simulink model "DDMR_SS"  (R2024b)
settings: Solver=VariableStepAuto  StartTime=0.0  StopTime=30  RelTol=1e-3
values from neighbouring files (symbols this model uses):
  A_steer = [0, -V_ref; 0, 0]    [LQR.m]    (also in Track.m; Track2.m)
  B_steer = [0; 1]    [LQR.m]    (also in Track.m; Track2.m)
  K = lqr(A_full, B_full, Q_lqr, R_lqr)    [LQR.m]    (also in Track.m = [K_brake, 0, 0; Track2.m)
  L = 0.2    [LQR.m]    (also in Track.m; Track2.m)
  L_f = 0.2    [LQR.m]    (also in Track.m; Track2.m)
  L_obs = lqr(A_steer', C_steer', Q_obs, R_obs)'    [LQR.m]    (also in Track.m = place(A_steer', C_steer', poles_obs)'; Track2.m)
  line_width = 0.03    [LQR.m]    (also in Track.m; Track2.m)
  R = 0.05    [LQR.m]    (also in Track.m; Track2.m)
  track_pts = [2*cos(linspace(0, 2*pi, 1000)'), 2*sin(linspace(0, 2*pi, 1000)').*cos(linspace(0, 2*pi, 1000)')]    [LQR.m]    (also in Track.m; Track2.m = [track_pts; segments{i}])
  W_spread = 0.15    [LQR.m]    (also in Track.m; Track2.m)
settings Model: Creator=moham  LastModifiedBy=moham

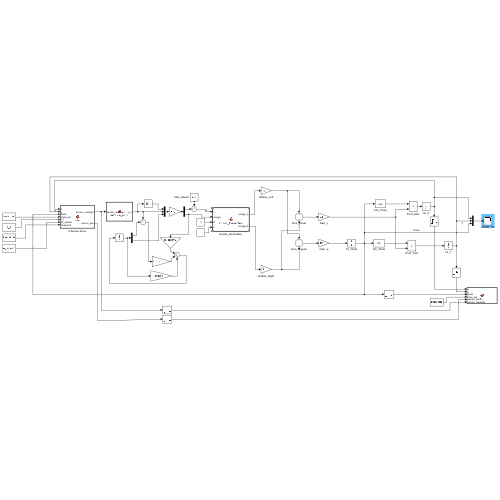
[thumbnail: Simulink's stored preview of the top-level diagram]
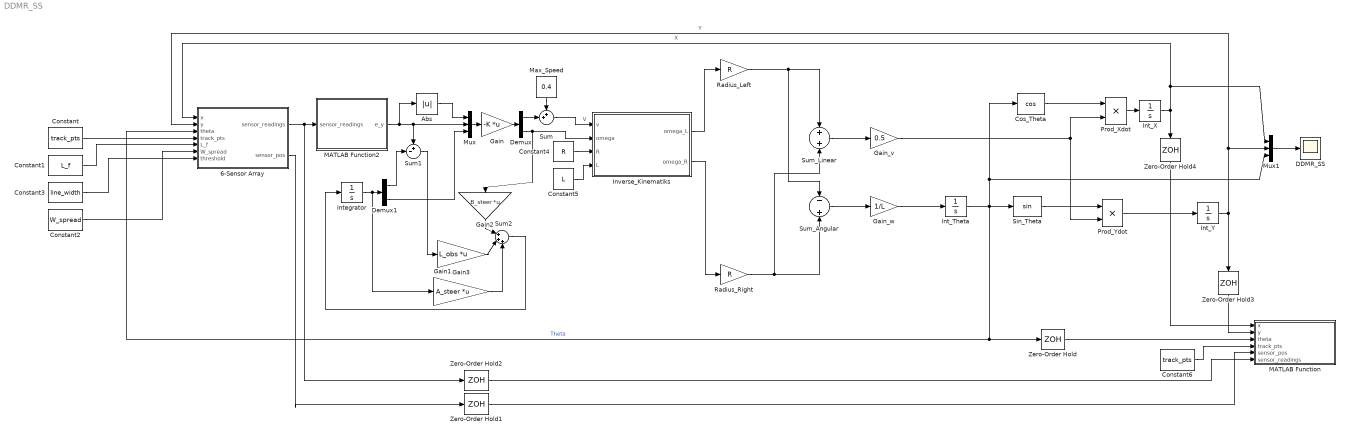
== system DDMR_SS ==
  6-Sensor Array : MATLAB Function  TreatAsAtomicUnit=on
  Abs : Abs  SaturateOnIntegerOverflow=off
  Constant : Constant  Value=track_pts
  Constant1 : Constant  Value=L_f
  Constant2 : Constant  Value=W_spread
  Constant3 : Constant  Value=line_width
  Constant4 : Constant  Value=R
  Constant5 : Constant  Value=L
  Constant6 : Constant  Value=track_pts
  Cos_Theta : Trigonometry  Operator=cos
  DDMR_SS : Scope
  Demux : Demux  Outputs=2
  Demux1 : Demux  Outputs=2
  Gain : Gain  Gain=-K  Multiplication=Matrix(K*u)
  Gain1 : Gain  Gain=A_steer  Multiplication=Matrix(K*u)
  Gain2 : Gain  Gain=B_steer  Multiplication=Matrix(K*u)
  Gain3 : Gain  Gain=L_obs  Multiplication=Matrix(K*u)
  Gain_v : Gain  Gain=0.5
  Gain_w : Gain  Gain=1/L
  Int_Theta : Integrator  InitialCondition=pi/-3
  Int_X : Integrator
  Int_Y : Integrator
  Integrator : Integrator  InitialCondition=[0; 0]
  "Inverse_Kinematiks " : MATLAB Function  TreatAsAtomicUnit=on
  MATLAB Function : MATLAB Function  TreatAsAtomicUnit=on
  MATLAB Function2 : MATLAB Function  TreatAsAtomicUnit=on
  Max_Speed : Constant  Value=0.4
  Mux : Mux  Inputs=3
  Mux1 : Mux  Inputs=3
  Prod_Xdot : Product
  Prod_Ydot : Product
  Radius_Left : Gain  Gain=R
  Radius_Right : Gain  Gain=R
  Sin_Theta : Trigonometry
  Sum : Sum  Inputs=++|
  Sum1 : Sum  Inputs=+-|
  Sum2 : Sum  Inputs=|+++
  Sum_Angular : Sum  Inputs=-+
  Sum_Linear : Sum
  Zero-Order Hold{,1..4} (5 alike) : ZeroOrderHold  SampleTime=0.033
  wires:
  "Inverse_Kinematiks "/1(omega_L) -> Radius_Left/1
  "Inverse_Kinematiks "/2(omega_R) -> Radius_Right/1
  Prod_Ydot/1 -> Int_Y/1
  Cos_Theta/1 -> Prod_Xdot/1
  Gain_v/1 -> Prod_Xdot/2, Prod_Ydot/2
  Sin_Theta/1 -> Prod_Ydot/1
  Prod_Xdot/1 -> Int_X/1
  Gain_w/1 -> Int_Theta/1
  Radius_Left/1 -> Sum_Linear/1, Sum_Angular/1
  Sum_Angular/1 -> Gain_w/1
  Radius_Right/1 -> Sum_Linear/2, Sum_Angular/2
  Sum_Linear/1 -> Gain_v/1
  Constant/1 -> 6-Sensor Array/4(track_pts)
  Constant1/1 -> 6-Sensor Array/5(L_f)
  Constant2/1 -> 6-Sensor Array/6(W_spread)
  Constant3/1 -> 6-Sensor Array/7(threshold)
  6-Sensor Array/1(sensor_readings) -> Zero-Order Hold2/1, MATLAB Function2/1(sensor_readings)
  MATLAB Function2/1(e_y) -> Sum1/1, Mux/2, Abs/1
  Sum/1 -> "Inverse_Kinematiks "/1(v)  "V"
  Constant4/1 -> "Inverse_Kinematiks "/3(R)
  Constant5/1 -> "Inverse_Kinematiks "/4(L)
  Constant6/1 -> MATLAB Function/4(track_pts)
  6-Sensor Array/2(sensor_pos) -> Zero-Order Hold1/1
  Zero-Order Hold1/1 -> MATLAB Function/5(sensor_pos)
  Zero-Order Hold2/1 -> MATLAB Function/6(sensor_readings)
  Zero-Order Hold/1 -> MATLAB Function/3(theta)
  Zero-Order Hold3/1 -> MATLAB Function/2(y)
  Zero-Order Hold4/1 -> MATLAB Function/1(x)
  Gain/1 -> Demux/1
  Demux/2 -> Gain2/1, "Inverse_Kinematiks "/2(omega)
  Demux/1 -> Sum/2
  Max_Speed/1 -> Sum/1
  Abs/1 -> Mux/1
  Mux/1 -> Gain/1
  Integrator/1 -> Gain1/1, Demux1/1
  Demux1/2 -> Mux/3
  Demux1/1 -> Sum1/2
  Gain3/1 -> Sum2/2
  Gain1/1 -> Sum2/3
  Gain2/1 -> Sum2/1
  Sum1/1 -> Gain3/1
  Sum2/1 -> Integrator/1
  Int_Theta/1 -> Sin_Theta/1, Zero-Order Hold/1, 6-Sensor Array/3(theta), Mux1/3, Cos_Theta/1  "Theta"
  Mux1/1 -> DDMR_SS/1
  Int_Y/1 -> 6-Sensor Array/2(y), Mux1/2, Zero-Order Hold3/1  "Y"
  Int_X/1 -> Mux1/1, 6-Sensor Array/1(x), Zero-Order Hold4/1  "X"

== matlab function DDMR_SS/MATLAB Function ==
  settings: updateMethod=DISCRETE
  data: x input; y input; theta input; track_pts input; sensor_pos input; sensor_readings input
function fcn(x, y, theta, track_pts, sensor_pos, sensor_readings)
    coder.extrinsic('figure', 'plot', 'hold', 'scatter', 'drawnow', 'gca', 'cla', 'axis', 'grid', 'ishandle', 'xlim', 'ylim');
    
    persistent fig;
    
    if isempty(fig)
        fig = figure('Name', '6-Sensor DDMR');
    elseif ~ishandle(fig)
        fig = figure('Name', '6-Sensor DDMR');
    end
    
    figure(fig); 
    ax = gca; 
    cla(ax); 
    hold(ax, 'on');
    
    % Draw Track
    plot(ax, track_pts(:,1), track_pts(:,2), 'k--', 'LineWidth', 2);
    
    % Draw Robot (Scaled to fit your L = 0.2m physical track width)
    R_chassis = 0.12; 
    th = linspace(0, 2*pi, 50);
    plot(ax, x + R_chassis*cos(th), y + R_chassis*sin(th), 'b', 'LineWidth', 1.5);
    
    % Plot heading line (Starts at the chassis edge, extends past the sensors to 0.3m)
    Pointer_L = 0.3; 
    plot(ax, [x + R_chassis*cos(theta), x + Pointer_L*cos(theta)], ...
             [y + R_chassis*sin(theta), y + Pointer_L*sin(theta)], 'r', 'LineWidth', 2);
    
    % Draw 6 Sensors (Red = off line, Green = on line)
    for i = 1:6
        c = 'r'; 
        if sensor_readings(i) == 1
            c = 'g'; 
        end
        scatter(ax, sensor_pos(1, i), sensor_pos(2, i), 40, c, 'filled');
    end
    
    % Dynamic sliding camera fix
    axis(ax, 'equal'); 
    xlim(ax, [x - 0.8, x + 0.8]);
    ylim(ax, [y - 0.8, y + 0.8]);
    
    grid(ax, 'on'); 
    hold(ax, 'off'); 
    drawnow;
end

== matlab function DDMR_SS/6-Sensor Array ==
  data: x input; sensor_readings output; y input; theta input; track_pts input; L_f input; W_spread input; threshold input; sensor_pos output
function [sensor_readings, sensor_pos] = fcn(x, y, theta, track_pts, L_f, W_spread, threshold)
    % 6 sensors spread linearly across the front
    y_offsets = linspace(W_spread/2, -W_spread/2, 6);
    S_loc = [L_f * ones(1,6); y_offsets];
    
    R = [cos(theta), -sin(theta); sin(theta), cos(theta)];
    
    sensor_pos = zeros(2, 6);
    sensor_readings = zeros(1, 6);
    
    for i = 1:6
        % Calculate global position of each sensor
        sensor_pos(:, i) = [x; y] + R * S_loc(:, i);
        
        % Check distance to the track
        dists = sqrt((track_pts(:,1) - sensor_pos(1, i)).^2 + (track_pts(:,2) - sensor_pos(2, i)).^2);
        if min(dists) <= threshold
            sensor_readings(i) = 1;
        end
    end
end

== matlab function DDMR_SS/MATLAB Function2 ==
  settings: updateMethod=DISCRETE
  data: sensor_readings input; e_y output
function e_y = calculate_error(sensor_readings)
    % Physical distances of each sensor from the center of the chassis (in meters)
    % Array total width = 0.15m (+/- 0.075m)
    weights = [0.075, 0.045, 0.015, -0.015, -0.045, -0.075]; 
    
    % Calculate physical lateral error (e_y) in meters
    if sum(sensor_readings) == 0
        e_y = 0; % Maintain heading if no line is detected
    else
        e_y = sum(sensor_readings .* weights);
    end
end

== matlab function DDMR_SS/Inverse_Kinematiks  ==
  data: v input; omega_L output; omega input; R input; L input; omega_R output
function [omega_L, omega_R] = inverse_kinematics(v, omega, R, L)
    % Calculate linear velocity of each wheel (m/s)
    v_L = v - (omega * L / 2);
    v_R = v + (omega * L / 2);

    % Convert linear velocity to angular velocity (rad/s)
    omega_L = v_L / R;
    omega_R = v_R / R;
end
